simulink model "finals"  (R2025b)
settings: Solver=FixedStepAuto  StartTime=0.0  StopTime=3600  RelTol=1e-3
undefined symbols (not defined in the file or in its folder): DiscIntNeverNeededParam
libraries: sim3dlib x1, sim3dautolib x1
settings Model: Creator=Mohamed  LastModifiedBy=Mohamed

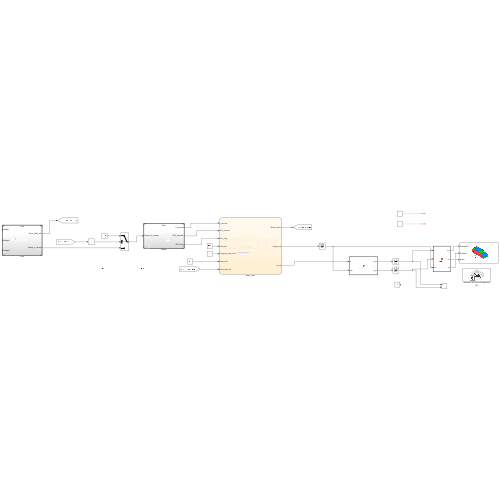
[thumbnail: Simulink's stored preview of the top-level diagram]
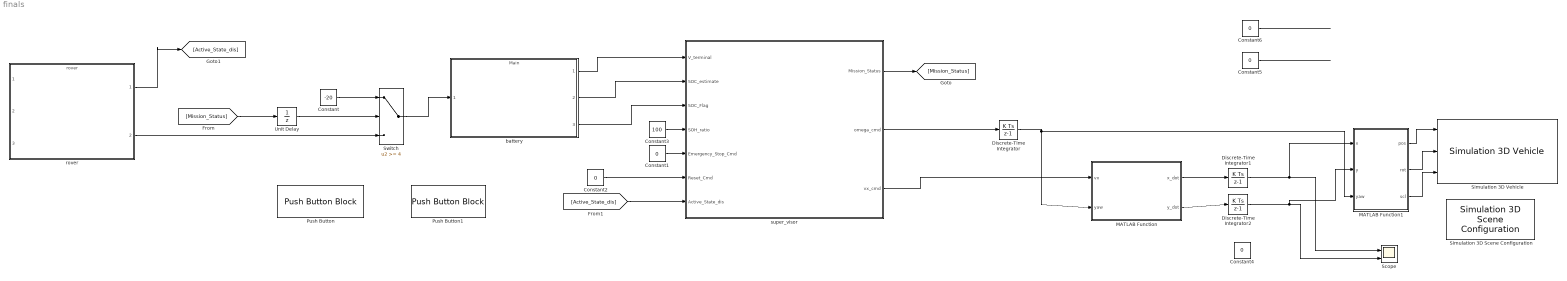
== system finals ==
  Constant : Constant  Value=-20
  Constant{1..2,4..6} (5 alike) : Constant  Value=0
  Constant3 : Constant  Value=100
  Discrete-Time Integrator : DiscreteIntegrator  SampleTime=-1  ICPrevOutput=DiscIntNeverNeededParam  ICPrevScaledInput=DiscIntNeverNeededParam
  Discrete-Time Integrator1 : DiscreteIntegrator  SampleTime=-1  ICPrevOutput=DiscIntNeverNeededParam  ICPrevScaledInput=DiscIntNeverNeededParam
  Discrete-Time Integrator2 : DiscreteIntegrator  SampleTime=-1  ICPrevOutput=DiscIntNeverNeededParam  ICPrevScaledInput=DiscIntNeverNeededParam
  MATLAB Function : MATLAB Function  TreatAsAtomicUnit=on
  MATLAB Function1 : MATLAB Function  TreatAsAtomicUnit=on
  Push Button : PushButtonBlock  ButtonText=Rest  IconOnColor=[0.0, 0.39215686274509803, 0.0]  IconOffColor=[0.0, 1.0, 0.0]  OffValue=1.000000
  Push Button1 : PushButtonBlock  ButtonText=stop  IconOnColor=[0.0, 0.39215686274509803, 0.0]  IconOffColor=[0.0, 1.0, 0.0]  OffValue=1.000000
  Scope : Scope  NumInputPorts=2
  Simulation 3D Scene Configuration : sim3dlib/Simulation 3D Scene Configuration  Priority=0  ProjectFormat=Default Scenes  SceneDesc=Airport  ProjectName=C:\Program Files\MATLAB\R2025b\toolbox\shared\sim3d_projects\automotive_project_windows\UE\WindowsNoEditor\VehicleSimulation.exe  ScenePath=/Game/Maps/HwStrght  EnableOpenDRIVE=off  vehTagList={'Custom';'Scene Origin';'SimulinkVehicle1'}  vehTag=SimulinkVehicle1  AttachedCameraRelativeTranslation=[0 0 0]  FreeCameraDefaultInitialTranslation=[-6, 0, 2]  AttachedCameraRelativeRotation=[0 0 0]  FreeCameraDefaultInitialRotation=[0, -15, 0]  ViewpointName=Custom  FreeCameraInitialTranslation=[-6, 0, 2]  ViewpointTranslation=[0 0 0]  FreeCameraInitialRotation=[0, -15, 0]  ViewpointRotation=[0 0 0]  OpVisEn=off  Ts=.02  EnableWindow=on  EnableRemoteAccess=off  EnableWeather=off  SunAzimuth=90  SunAltitude=40.0  EnableGeospatialSun=off  Latitude=0  Longitude=0  Date=2023-01-01  Time=10:30:00  GeoTimeZone=-5.0  SunDaylightSaving=off  wind=1  clouds=10  EnableVolumetricClouds=off  CloudCoverage=0  CloudAltitude=6  fog=0  rain=0  RaindropsEffect=off  SnowDensity=0  EnableGeospatial=off  TilesetSource=Earth terrain  UseTrueOrigin=off  OriginHeight=200  OriginLatitude=40.744652  OriginLongitude=-73.988864  MapStyle=Aerial  AdditionalAssetIDs=[]  UseAdvancedSunSky=off  SolarTime=11  TimeZone=-5  Day=21  Month=9  Year=2022  UseDaylightSavingTime=on  DSTStartDay=10  DSTStartMonth=3  DSTEndDay=3  DSTEndMonth=11  DSTSwitchHour=2  sensorTag=MainCamera1  sensorId=1  sensorName=MainCamera1  mountLoc=Origin  offsetFlag=off  tmountOffset=[0, 0, 0]  rmountOffset=[0, 0, 0]  HorizontalResolution=1280  VerticalResolution=720  HorizontalFOV=60  mountPoint=[0 0 0]  mountOrientation=[0 0 0]  aMode=0  ID=1  GeoTrigger=Inactive  ViewNameList={'Custom'}  ViewTranslationList={'[-6 0 2]'}  ViewRotationList={'[0 -15 0]'}
      settings: AttributesFormatString=NED  LibrarySourceBlock=aerolibsim3d/Simulation 3D Scene Configuration
  Simulation 3D Vehicle : sim3dautolib/Simulation 3D Vehicle  Priority=-1  PassVehMesh=Muscle car  MeshPath=/MathWorksAutomotiveContent/Vehicles/Muscle/Meshes/SK_MuscleCar.SK_MuscleCar  VehColor=Red  ActorName=SimulinkVehicle1  VehLightsControl=off  HeadlightColor=[ 1, 1, 1 ]  HighBeamIntensity=100000  LowBeamIntensity=60000  HighBeamConeAngle=1.22  LowBeamConeAngle=1.22  LeftHeadlightOrientation=[ 0, 0 ]  RightHeadlightOrientation=[ 0, 0 ]  BrakelightIntensity=500  ReverselightIntensity=500  SignallightIntensity=500  SignallightPeriod=1  SignalPulseWidth=50  Translation=zeros( 5, 3 )  Rotation=zeros( 5, 3 )  Scale=ones( 5, 3 )  SampleTime=-1  ActorType=SimulinkVehicle  ID=1  aMode=2  ActorTag=SimulinkVehicle1
      settings: LibrarySourceBlock=vehdynlibsim3d/Simulation 3D Vehicle
  Switch : Switch  Threshold=4  SaturateOnIntegerOverflow=off  InputSameDT=off
  Unit Delay : UnitDelay  SampleTime=-1  HasFrameUpgradeWarning=on
  battery : ModelReference  ModelNameDialog=Main.slx  SimulationMode=Normal  ModelReferenceVersion=1.8
  rover : ModelReference  ModelNameDialog=rover.slx  SimulationMode=Normal  ModelReferenceVersion=1.12
  super_visor : Stateflow chart  TreatAsAtomicUnit=on
      settings: PortSchema="{\"entries\":[{\"content\":{\"sides\":[{\"content\":{\"connectorIds\":[\"In2\",\"In1\",\"In3\",\"In4\",\"In5\",\"In6\",\"In7\"]},\"type\":\"ConnectorPlacement.EquallySpacedRectSide\",\"uuid\":\"a466a9a6-c2b2-4fcb-9285-f02016f0e773\"},{\"content\":{\"connectorIds\":[\"Out1\",\"Out2\",\"Out3\"],\"side\":\"RIGHT\"},\"type\":\"ConnectorPlacement.EquallySpacedRectSide\",\"uuid\":\"662d6096-1f3f-4662-af24-506c775b1a2d\"},{\"content\":{\"side\":\"TOP\"},\"type\":\"ConnectorPlacement.EquallySpacedRectSide\",\"uuid\":\"e501738c-616a-43f4-a44f-0cc0624f093c\"}]},\"type\":\"ConnectorPlacement.EquallySpacedConnector\",\"uuid\":\"34257f68-8411-42c1-86e4-70195f026b45\"}],\"packageUris\":[\"http://schema.mathworks.com/mf0/Connector/R2020b\"],\"version\":\"1.0\"}"
  wires:
  battery/3 -> super_visor/3(SOC_Flag)
  battery/2 -> super_visor/1(SOC_estimate)
  battery/1 -> super_visor/2(V_terminal)
  Switch/1 -> battery/1
  Constant/1 -> Switch/1
  rover/2 -> Switch/3
  super_visor/1(Mission_Status) -> [Mission_Status]
  [Mission_Status] -> Unit Delay/1
  Unit Delay/1 -> Switch/2
  Constant2/1 -> super_visor/6(Reset_Cmd)
  Constant1/1 -> super_visor/5(Emergency_Stop_Cmd)
  rover/1 -> [Active_State_dis]
  [Active_State_dis] -> super_visor/7(Active_State_dis)
  Constant3/1 -> super_visor/4(SOH_ratio)
  super_visor/2(omega_cmd) -> Discrete-Time Integrator/1
  super_visor/3(vx_cmd) -> MATLAB Function/1(vx)
  Discrete-Time Integrator/1 -> MATLAB Function1/3(yaw), MATLAB Function/2(yaw)
  MATLAB Function/2(y_dot) -> Discrete-Time Integrator2/1
  MATLAB Function/1(x_dot) -> Discrete-Time Integrator1/1
  Discrete-Time Integrator1/1 -> MATLAB Function1/1(x), Scope/1
  Discrete-Time Integrator2/1 -> MATLAB Function1/2(y), Scope/2
  Constant5/1 -> ?
  Constant6/1 -> ?
  MATLAB Function1/1(pos) -> Simulation 3D Vehicle/1
  MATLAB Function1/2(rot) -> Simulation 3D Vehicle/2
  MATLAB Function1/3(scl) -> Simulation 3D Vehicle/3

== matlab function finals/MATLAB Function1 ==
  data: x input; pos output; y input; yaw input; rot output; scl output
function [pos, rot, scl] = pack_3d(x, y, yaw)
    % Row 1 is the car body (it gets the real coordinates)
    % Rows 2-5 are the wheels (0 offset keeps them attached to the car)
    pos = [x, y, 0;
           0, 0, 0;
           0, 0, 0;
           0, 0, 0;
           0, 0, 0];
    
    rot = [0, 0, yaw;
           0, 0, 0;
           0, 0, 0;
           0, 0, 0;
           0, 0, 0];
           
    % Scale remains 1 for all parts so they don't disappear
    scl = [1, 1, 1;
           1, 1, 1;
           1, 1, 1;
           1, 1, 1;
           1, 1, 1];
end

== matlab function finals/MATLAB Function ==
  data: vx input; x_dot output; yaw input; y_dot output
function [x_dot, y_dot] = get_XY_vel(vx, yaw)
x_dot = vx * cos(yaw);
y_dot = vx * sin(yaw);

== stateflow chart finals/super_visor ==
  state operating
    state nominal
      en: Mission_Status = 1;
      du: [vx_cmd, omega_cmd] = StateToKinematics(Active_State_dis, 1.0, 1.0);
    state low_power
      en: Mission_Status = 2;
      du: [vx_cmd, omega_cmd] = StateToKinematics(Active_State_dis, 0.5, 0.5);
    state cell_fault
      en: Mission_Status = 3;
      du: [vx_cmd, omega_cmd] = StateToKinematics(Active_State_dis, 0.2, 0.2);
    (default) -> nominal
    nominal -> low_power [order 2] : [SOC_estimate < 20 || SOH_ratio < 80]
    nominal -> cell_fault [order 1] : [SOC_Flag == true]
    cell_fault -> nominal : [SOC_Flag == false]
    low_power -> nominal : [SOC_estimate >= 20 && SOH_ratio >= 80]
  state return_to_base
    en: Mission_Status = 4;
    vx_cmd = 0;
    omega_cmd = 0;
  (default) -> operating
  operating -> return_to_base [order 2] : [Emergency_Stop_Cmd == true]
  operating -> return_to_base [order 1] : [SOC_estimate < 5 || V_terminal < 2.5]
  return_to_base -> operating : [Reset_Cmd == true]
  data: state function_input; vx_scale function_input; omega_scale function_input; vx function_output; omega function_output; Mission_Status output; omega_cmd output; vx_cmd output; SOC_estimate input; V_terminal input; SOC_Flag input; SOH_ratio input; Emergency_Stop_Cmd input; Reset_Cmd input; Active_State_dis input
  function [vx, omega] = StateToKinematics(state, vx_scale, omega_scale):
    | function [vx, omega] = StateToKinematics(state, vx_scale, omega_scale)
    |  
    | if state == 1
    |     vx = 2.0 * vx_scale;
    |     omega = 0.0;
    | elseif state == 2
    |     vx = 0.0;
    |     omega = 1.0 * omega_scale;
    | elseif state == 3
    |     vx = 0.0;
    |     omega = -1.0 * omega_scale;
    | else
    |     % Covers 0 (IDLE) and 4 (STOP)
    |     vx = 0.0;
    |     omega = 0.0;
    | end
